simulink model "ContBasZEnvioTodo"  (R2026b)
settings: Solver=FixedStepAuto  StopTime=inf  EnableMultiTasking=on
libraries: px4uORBlib x5, px4Peripheralslib x2
settings Model: Creator=cfmm  LastModifiedBy=cfmm
settings SolverCC: PositivePriorityOrder=on
settings OptimizationCC: DifferentSizesBufferReuse=on  EfficientTunableParamExpr=on  EnhancedBackFolding=on  MaxStackSize=64  OptimizationCustomize=off  OptimizeBlockOrder=speed  PassReuseOutputArgsAs=Individual arguments  RemoveInternalMemoryZeroInit=on  RemoveRootLevelIOMemoryZeroInit=on
settings DebuggingCC: ParameterTunabilityLossMsg=error
settings HardwareCC: ProdHWDeviceType=ARM Compatible->ARM Cortex  ProdLargestAtomicFloat=Double  ProdLargestAtomicInteger=Long  ProdLongLongMode=on
settings SFSimCC: MATLABDynamicMemAlloc=off  SimTargetLang=C++
settings RTWCC: Description=Embedded Coder  HardwareBoard=PX4 Host Target  PortableWordSizes=on  SystemTargetFile=ert.tlc  TLCOptions="-aInlineSetEventsForThisBaseRateFcn=TLC_FALSE -aSuppressMultiTaskScheduler=TLC_FALSE  -aRateBasedStepFcn=0"  TargetLang=C++  TemplateMakefile=ert_default_tmf  Toolchain=GNU Tools for PX4 Autopilots
settings CodeAppCC: ForceParamTrailComments=on  IgnoreCustomStorageClasses=off  InsertBlockDesc=on  OperatorAnnotations=on  SFDataObjDesc=on  SimulinkDataObjDesc=on
settings ERTTargetCC: CombineSignalStateStructs=on  ExtModeIntrfLevel=Level2 - Open  ExtModeMexFile=ext_xcp  ExtModeStaticAlloc=on

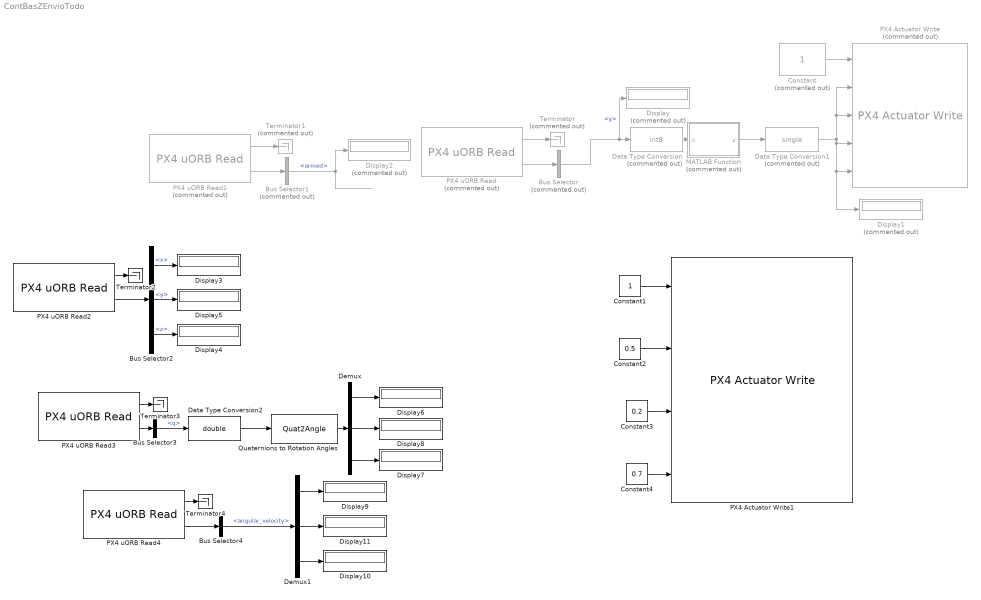
== system ContBasZEnvioTodo ==
  Bus Selector : BusSelector  Commented=on  OutputSignals=y
  Bus Selector1 : BusSelector  Commented=on  OutputSignals=armed
  Bus Selector2 : BusSelector  OutputSignals=x,y,z
  Bus Selector3 : BusSelector  OutputSignals=q
  Bus Selector4 : BusSelector  OutputSignals=angular_velocity
  Constant : Constant  Commented=on  OutDataTypeStr=boolean
  Constant1 : Constant  OutDataTypeStr=boolean
  Constant2 : Constant  Value=0.5  OutDataTypeStr=single  SampleTime=0.01
  Constant3 : Constant  Value=0.2  OutDataTypeStr=single  SampleTime=0.01
  Constant4 : Constant  Value=0.7  OutDataTypeStr=single  SampleTime=0.01
  Data Type Conversion : DataTypeConversion  Commented=on  OutDataTypeStr=int8  SaturateOnIntegerOverflow=off  RndMeth=Floor
  Data Type Conversion1 : DataTypeConversion  Commented=on  OutDataTypeStr=single  SaturateOnIntegerOverflow=off  RndMeth=Floor
  Data Type Conversion2 : DataTypeConversion  OutDataTypeStr=double  SaturateOnIntegerOverflow=off  RndMeth=Floor
  Demux : Demux  Outputs=3
  Demux1 : Demux  Outputs=3
  Display : Display  Commented=on
  Display1 : Display  Commented=on
  Display{3..11} (9 alike) : Display
  Display2 : Display  Commented=on
  MATLAB Function : MATLAB Function  Commented=on  TreatAsAtomicUnit=on
  PX4 Actuator Write : px4Peripheralslib/PX4 Actuator Write  Commented=on  Motor1Enable=on  Motor2Enable=on  Motor3Enable=on  Motor4Enable=on  Motor5Enable=off  Motor6Enable=off  Motor7Enable=off  Motor8Enable=off  Motor9Enable=off  Motor10Enable=off  Motor11Enable=off  Motor12Enable=off  IsMotorArray=off  Servo1Enable=off  Servo2Enable=off  Servo3Enable=off  Servo4Enable=off  Servo5Enable=off  Servo6Enable=off  Servo7Enable=off  Servo8Enable=off  IsServoArray=off
  PX4 Actuator Write1 : px4Peripheralslib/PX4 Actuator Write  Motor1Enable=on  Motor2Enable=on  Motor3Enable=on  Motor4Enable=off  Motor5Enable=off  Motor6Enable=off  Motor7Enable=off  Motor8Enable=off  Motor9Enable=off  Motor10Enable=off  Motor11Enable=off  Motor12Enable=off  IsMotorArray=off  Servo1Enable=off  Servo2Enable=off  Servo3Enable=off  Servo4Enable=off  Servo5Enable=off  Servo6Enable=off  Servo7Enable=off  Servo8Enable=off  IsServoArray=off
  PX4 uORB Read : px4uORBlib/PX4 uORB Read  Commented=on  uORBMsg=SensorGyro  uORBTopicName=sensor_gyro  SubscribeNonZeroInstance=off  selectInstanceNum=1  SampleTime=0.01  isSingleTopicMsg=on  BlockingMode=off  BlockTimeout=1e-3
  PX4 uORB Read1 : px4uORBlib/PX4 uORB Read  Commented=on  uORBMsg=ActuatorArmed  uORBTopicName=actuator_armed  SubscribeNonZeroInstance=off  selectInstanceNum=1  SampleTime=0.01  isSingleTopicMsg=on  BlockingMode=off  BlockTimeout=1e-3
  PX4 uORB Read2 : px4uORBlib/PX4 uORB Read  uORBMsg=VehicleLocalPosition  uORBTopicName=vehicle_local_position  SubscribeNonZeroInstance=off  selectInstanceNum=1  SampleTime=0.01  isSingleTopicMsg=off  BlockingMode=off  BlockTimeout=1e-3
  PX4 uORB Read3 : px4uORBlib/PX4 uORB Read  uORBMsg=VehicleAttitude  uORBTopicName=vehicle_attitude  SubscribeNonZeroInstance=off  selectInstanceNum=1  SampleTime=0.01  isSingleTopicMsg=off  BlockingMode=off  BlockTimeout=1e-3
  PX4 uORB Read4 : px4uORBlib/PX4 uORB Read  uORBMsg=VehicleOdometry  uORBTopicName=vehicle_odometry  SubscribeNonZeroInstance=off  selectInstanceNum=1  SampleTime=0.01  isSingleTopicMsg=off  BlockingMode=off  BlockTimeout=1e-3
  Quaternions to Rotation Angles : Quat2Angle
      settings: AttributesFormatString=Rotation Order: %<rotationOrder>
  Terminator : Terminator  Commented=on
  Terminator1 : Terminator  Commented=on
  Terminator2 : Terminator
  Terminator3 : Terminator
  Terminator4 : Terminator
  wires:
  Bus Selector1/1 -> Display2/1  "<armed>"
  MATLAB Function/1(y) -> Data Type Conversion1/1
  PX4 uORB Read/2 -> Bus Selector/1
  Bus Selector/1 -> Data Type Conversion/1, Display/1  "<y>"
  Data Type Conversion/1 -> MATLAB Function/1(u)
  Data Type Conversion1/1 -> PX4 Actuator Write/4, PX4 Actuator Write/5, Display1/1, PX4 Actuator Write/3, PX4 Actuator Write/2
  PX4 uORB Read/1 -> Terminator/1
  PX4 uORB Read1/1 -> Terminator1/1
  PX4 uORB Read1/2 -> Bus Selector1/1
  Constant/1 -> PX4 Actuator Write/1
  PX4 uORB Read2/1 -> Terminator2/1
  PX4 uORB Read3/1 -> Terminator3/1
  PX4 uORB Read4/1 -> Terminator4/1
  PX4 uORB Read2/2 -> Bus Selector2/1
  PX4 uORB Read3/2 -> Bus Selector3/1
  PX4 uORB Read4/2 -> Bus Selector4/1
  Bus Selector3/1 -> Data Type Conversion2/1  "<q>"
  Bus Selector2/1 -> Display3/1  "<x>"
  Bus Selector2/3 -> Display4/1  "<z>"
  Bus Selector2/2 -> Display5/1  "<y>"
  Quaternions to Rotation Angles/1 -> Demux/1
  Demux/2 -> Display8/1
  Demux/3 -> Display7/1
  Demux/1 -> Display6/1
  Bus Selector4/1 -> Demux1/1  "<angular_velocity>"
  Demux1/2 -> Display11/1
  Demux1/1 -> Display9/1
  Demux1/3 -> Display10/1
  Constant1/1 -> PX4 Actuator Write1/1
  Data Type Conversion2/1 -> Quaternions to Rotation Angles/1
  Constant2/1 -> PX4 Actuator Write1/2
  Constant3/1 -> PX4 Actuator Write1/3
  Constant4/1 -> PX4 Actuator Write1/4

== matlab function ContBasZEnvioTodo/MATLAB Function ==
  data: u input; y output
function y = fcn(u)
if (u > 5)
    y = 0.1;
else
    y = 0.7;
end
